simulink model "sensor_real_corriente_LU"  (R2026b)
settings: Solver=VariableStepAuto
undefined symbols (not defined in the file): wn_I, zeta_I
settings Model: Creator=lamun  LastModifiedBy=fedeb

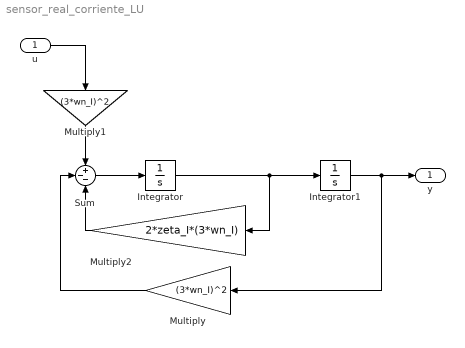
== system sensor_real_corriente_LU ==
  u : Inport
  Integrator : Integrator
  Integrator1 : Integrator
  Multiply : Gain  Gain=(3*wn_I)^2
  Multiply1 : Gain  Gain=(3*wn_I)^2
  Multiply2 : Gain  Gain=2*zeta_I*(3*wn_I)
  Sum : Sum  Inputs=+--
  y : Outport
  wires:
  Integrator/1 -> Multiply2/1, Integrator1/1
  Multiply1/1 -> Sum/1
  u/1 -> Multiply1/1
  Multiply2/1 -> Sum/3
  Sum/1 -> Integrator/1
  Multiply/1 -> Sum/2
  Integrator1/1 -> Multiply/1, y/1
